simulink model "ECP_SimplifiedInvertedPendulum"  (R2025a)
settings: Solver=VariableStepAuto  StartTime=0.0  StopTime=10.0  RelTol=1e-3
values from neighbouring files (symbols this model uses):
  den_g2 = [1 0 -(m_1*l_o+m_2*l_c)*g/J_oe]    [SlidingRodPendulum_Modeling.m]
  k_a = 2546    [SlidingRodPendulum_Modeling.m]
  k_hw = k_x*k_s*k_f    (= 2088.32)    [SlidingRodPendulum_Modeling.m]
  k_pfc = S0+R0/G2_dc    [SlidingRodPendulum_Modeling.m]
  k_s = 32    [SlidingRodPendulum_Modeling.m]
  k_star = (k_a*m_1*l_o)/(k_x*J_oe)    (= 0.059867860237)    [SlidingRodPendulum_Modeling.m]
  kd = 2*zeta*wn*m_star/k_hw    (= 0.00784530292237)    [SlidingRodPendulum_Modeling.m]
  kp = m_star*wn^2/k_hw    (= 0.247127042055)    [SlidingRodPendulum_Modeling.m]
  m_star = (m_1*m_2_star)/(m_1+m_2_star)    (= 0.130027801578)    [SlidingRodPendulum_Modeling.m]
  num_g2 = [-1 0 g/l_o]    [SlidingRodPendulum_Modeling.m]
  r_0_val = double(sol.r_0)    [SlidingRodPendulum_Modeling.m]
  r_1_val = double(sol.r_1)    [SlidingRodPendulum_Modeling.m]
  s_0_val = double(sol.s_0)    [SlidingRodPendulum_Modeling.m]
  s_1_val = double(sol.s_1)    [SlidingRodPendulum_Modeling.m]
libraries: slpidlib x1
settings Model: Creator=young  LastModifiedBy=young

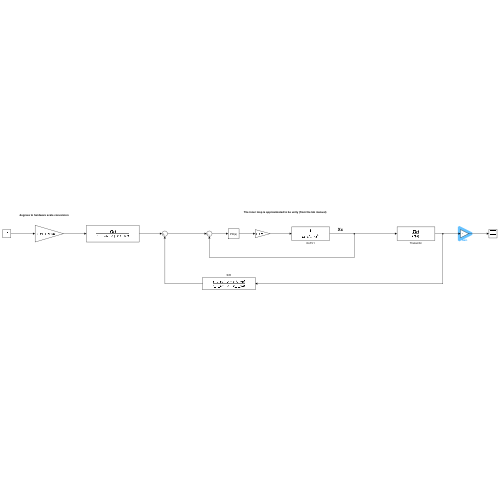
[thumbnail: Simulink's stored preview of the top-level diagram]
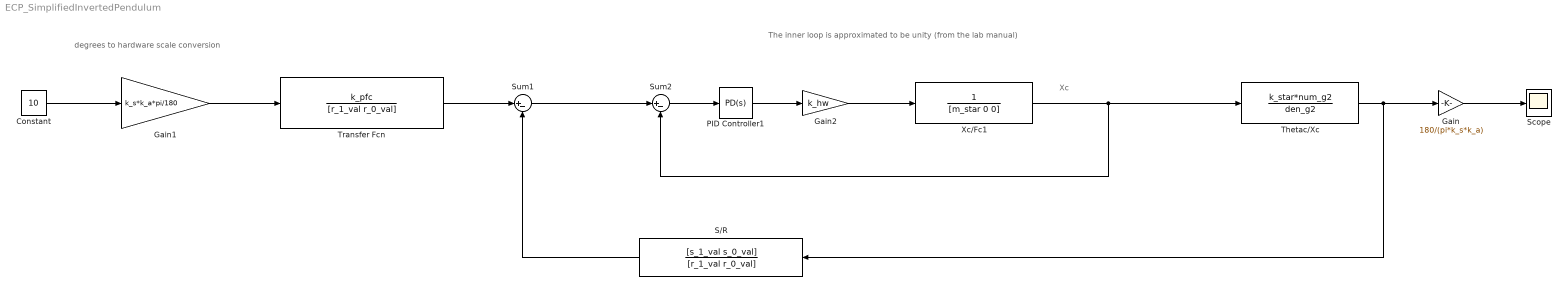
== system ECP_SimplifiedInvertedPendulum ==
  note: The inner loop is approximated to be unity (from the lab manual)
  note: degrees to hardware scale conversion
  note: Xc
  Constant : Constant  Value=10
  Gain : Gain  Gain=180/(pi*k_s*k_a)
  Gain1 : Gain  Gain=k_s*k_a*pi/180
  Gain2 : Gain  Gain=k_hw
  PID Controller1 : slpidlib/PID Controller  Controller=PD  Form=Parallel  TimeDomain=Continuous-time  UseExternalTs=off  SampleTime=-1  IntegratorMethod=Forward Euler  FilterMethod=Forward Euler  ControllerParametersSource=internal  P=kp  I=1  UseKiTs=off  D=kd  UseExternalDerivativeSource=off  N=100  UseFilter=on  TunerSelectOption=Transfer Function Based (PID Tuner App)  InitialConditionSource=internal  InitialConditionForIntegrator=0  InitialConditionForFilter=0  DifferentiatorICPrevScaledInput=0  ExternalReset=none  TrackingMode=off  Kt=1  LimitOutput=off  SatLimitsSource=internal  UpperSaturationLimit=inf  LowerSaturationLimit=-inf  LinearizeAsGain=on  AntiWindupMode=none  Kb=1  LimitIntegrator=off  UpperIntegratorSaturationLimit=inf  LowerIntegratorSaturationLimit=-inf  POutMin=[]  POutMax=[]  IOutMin=[]  IOutMax=[]  DOutMin=[]  DOutMax=[]  NOutMin=[]  NOutMax=[]  SumOutMin=[]  SumOutMax=[]  SaturationOutMin=[]  SaturationOutMax=[]  PParamMin=[]  PParamMax=[]  IParamMin=[]  IParamMax=[]  DParamMin=[]  DParamMax=[]  NParamMin=[]  NParamMax=[]  KbParamMin=[]  KbParamMax=[]  KtParamMin=[]  KtParamMax=[]  KbOutMin=[]  KbOutMax=[]  KtOutMin=[]  KtOutMax=[]  IntegratorOutMin=[]  IntegratorOutMax=[]  FilterOutMin=[]  FilterOutMax=[]  SumI1OutMin=[]  SumI1OutMax=[]  SumI2OutMin=[]  SumI2OutMax=[]  SumI3OutMin=[]  SumI3OutMax=[]  SumI4OutMin=[]  SumI4OutMax=[]  SumDOutMin=[]  SumDOutMax=[]  DifferentiatorOutMin=[]  DifferentiatorOutMax=[]  FilterDiffOutCoefMin=[]  FilterDiffOutCoefMax=[]  ReciprocalOutMin=[]  ReciprocalOutMax=[]  SumDenOutMin=[]  SumDenOutMax=[]  SumNumOutMin=[]  SumNumOutMax=[]  DivideOutMin=[]  DivideOutMax=[]  UdiffTsProdOutMin=[]  UdiffTsProdOutMax=[]  NTsProdOutMin=[]  NTsProdOutMax=[]  UintegralTsProdOutMin=[]  UintegralTsProdOutMax=[]  UngainTsProdOutMin=[]  UngainTsProdOutMax=[]  ClampingZeroOutDataTypeStr=Inherit: Inherit via back propagation  ClampingZeroOutMin=[]  ClampingZeroOutMax=[]  FilterDenConstantOutDataTypeStr=Inherit: Inherit via back propagation  FilterDenConstantOutMin=[]  FilterDenConstantOutMax=[]  PCopyOutDataTypeStr=Inherit: Inherit via back propagation  PCopyOutMin=[]  PCopyOutMax=[]  NCopyOutDataTypeStr=Inherit: Inherit via back propagation  NCopyOutMin=[]  NCopyOutMax=[]  IntegratorContinuousStateAttributes=''  IntegratorStateMustResolveToSignalObject=off  IntegratorRTWStateStorageClass=Auto  FilterContinuousStateAttributes=''  FilterStateMustResolveToSignalObject=off  FilterRTWStateStorageClass=Auto  ParallelPVariant=InternalParameters  IdealPVariant=Disabled  IVariant=Disabled  DVariant=InternalParameters  IntegratorVariant=Disabled  SatVariant=Disabled  AWVariant=Disabled  PCopyVariant=Disabled  TRVariant=Disabled  FdbkBlocksVariant=Forward  IdealPFdbkVariant=Disabled  SatFdbkVariant=Disabled  DerivativeFilterVariant=ContFilter  NVariant=InternalParameters  NCopyVariant=Disabled  FilterICVariant=InternalICsFilter  IntegratorICVariant=Disabled  ExternalResetVariant=Disabled  TRSumVariant=Passthrough  SumFdbkVariant=Disabled  SumVariant=Sum_PD  TsampFilterVariant=InternalTs  TsampNgainVariant=Passthrough  TsampIntegralVariant=Disabled_SignalSpec  ExternalSaturationOutDataTypeStr=Inherit: Same as second input  DerivativeSourceVariant=ErrorSignal  PreIntVariant=InternalPreInt
  S/R : TransferFcn  Numerator=[s_1_val s_0_val]  Denominator=[r_1_val r_0_val]
  Scope : Scope
      settings: ActiveDisplayYMinimum=-5.387830481176195  ActiveDisplayYMaximum=12.551609568178611
  Sum1 : Sum  Inputs=|+-
  Sum2 : Sum  Inputs=|+-
  Thetac/Xc : TransferFcn  Numerator=k_star*num_g2  Denominator=den_g2
  Transfer Fcn : TransferFcn  Numerator=k_pfc  Denominator=[r_1_val r_0_val]
  Xc/Fc1 : TransferFcn  Denominator=[m_star 0 0]
  wires:
  Transfer Fcn/1 -> Sum1/1
  Thetac/Xc/1 -> Gain/1, S/R/1
  S/R/1 -> Sum1/2
  Constant/1 -> Gain1/1
  Gain1/1 -> Transfer Fcn/1
  Gain2/1 -> Xc/Fc1/1
  Xc/Fc1/1 -> Thetac/Xc/1, Sum2/2
  PID Controller1/1 -> Gain2/1
  Sum2/1 -> PID Controller1/1
  Gain/1 -> Scope/1
  Sum1/1 -> Sum2/1
